simulink model "multimodecbf"  (R2025b)
settings: Solver=FixedStepAuto  StartTime=0.0  StopTime=inf  FixedStep=0.05  RelTol=1e-3
libraries: robotlib x14
settings Model: Creator=sprinkle  LastModifiedBy=sanborkl
settings OptimizationCC: DefaultParameterBehavior=Inlined  EnhancedBackFolding=on  PassReuseOutputArgsAs=Individual arguments  ZeroExternalMemoryAtStartup=off  ZeroInternalMemoryAtStartup=off  MaxStackSize=64  OptimizeBlockOrder=speed  DifferentSizesBufferReuse=on  OptimizationCustomize=off  EfficientTunableParamExpr=on
settings DebuggingCC: ParameterTunabilityLossMsg=error
settings HardwareCC: ProdBitPerPointer=32.0  ProdBitPerSizeT=32.0  ProdBitPerPtrDiffT=32.0  ProdLargestAtomicFloat=None  ProdIntDivRoundTo=Undefined  ProdEndianess=Unspecified  ProdWordSize=32.0  ProdHWDeviceType=Generic->Unspecified (assume 32-bit Generic)
settings SFSimCC: MATLABDynamicMemAlloc=off
settings RTWCC: SystemTargetFile=ert.tlc  HardwareBoard=Robot Operating System (ROS)  TLCOptions="-aInlineSetEventsForThisBaseRateFcn=TLC_FALSE -aSuppressMultiTaskScheduler=TLC_FALSE  -aRateBasedStepFcn=0"  GenCodeOnly=on  TemplateMakefile=ert_default_tmf  Toolchain=Catkin  TargetLang=C++  Description=Embedded Coder
settings CodeAppCC: ForceParamTrailComments=on  IgnoreCustomStorageClasses=off  OperatorAnnotations=on  SimulinkDataObjDesc=on  SFDataObjDesc=on  InsertBlockDesc=on

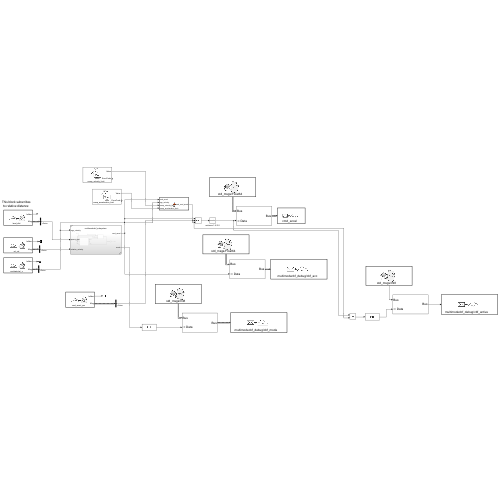
[thumbnail: Simulink's stored preview of the top-level diagram]
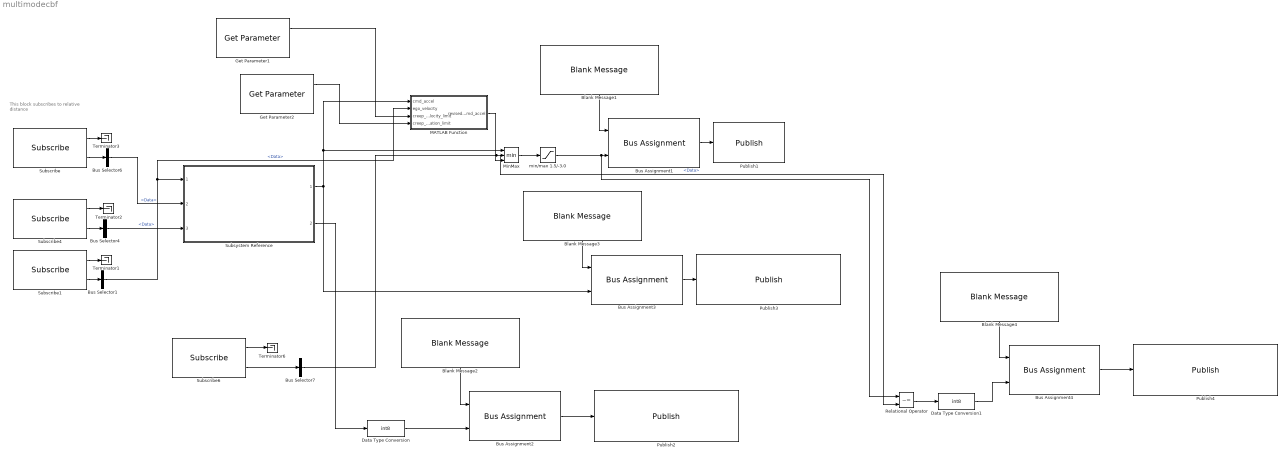
== system multimodecbf ==
  note: This block subscribes
      | to relative distance
  Blank Message1 : robotlib/Blank Message  messageClass=Message  entityType=std_msgs/Float64  messageType=std_msgs/Float64  SampleTime=inf  legacyBusStruct=off
  Blank Message2 : robotlib/Blank Message  messageClass=Message  entityType=std_msgs/Int8  messageType=std_msgs/Int8  SampleTime=inf  legacyBusStruct=off
  Blank Message3 : robotlib/Blank Message  messageClass=Message  entityType=std_msgs/Float64  messageType=std_msgs/Float64  SampleTime=inf  legacyBusStruct=off
  Blank Message4 : robotlib/Blank Message  messageClass=Message  entityType=std_msgs/Int8  messageType=std_msgs/Int8  SampleTime=inf  legacyBusStruct=off
  Bus Assignment{1..4} (4 alike) : BusAssignment  AssignedSignals=Data
  Bus Selector{1,4,6..7} (4 alike) : BusSelector  OutputSignals=Data
  Data Type Conversion : DataTypeConversion  OutDataTypeStr=int8  SaturateOnIntegerOverflow=off  RndMeth=Floor
  Data Type Conversion1 : DataTypeConversion  OutDataTypeStr=int8  SaturateOnIntegerOverflow=off  RndMeth=Floor
  Get Parameter1 : robotlib/Get Parameter  ParameterSource=Specify your own  ParameterName=creep_velocity_limit  ParameterType=double  ParameterMaxArrayLength=16  ParameterInitialValue=0.1  SampleTime=-1  ShowErrorCodeOutput=on  ModelName=multimodecbf  BlockId=ParamGet_multimodecbf_97
  Get Parameter2 : robotlib/Get Parameter  ParameterSource=Specify your own  ParameterName=creep_acceleration_limit  ParameterType=double  ParameterMaxArrayLength=16  ParameterInitialValue=0.0  SampleTime=-1  ShowErrorCodeOutput=on  ModelName=multimodecbf  BlockId=ParamGet_multimodecbf_98
  MATLAB Function : MATLAB Function  TreatAsAtomicUnit=on
  MinMax : MinMax  Inputs=3
  Publish1 : robotlib/Publish  topicSource=Specify your own  topic=cmd_accel  messageType=std_msgs/Float64  legacyBusStruct=off  messageQueueLength=1
  Publish2 : robotlib/Publish  topicSource=Specify your own  topic=multimodecbf_debug/cbf_mode  messageType=std_msgs/Int8  legacyBusStruct=off  messageQueueLength=1
  Publish3 : robotlib/Publish  topicSource=Specify your own  topic=multimodecbf_debug/cbf_acc  messageType=std_msgs/Float64  legacyBusStruct=off  messageQueueLength=1
  Publish4 : robotlib/Publish  topicSource=Specify your own  topic=multimodecbf_debug/cbf_active  messageType=std_msgs/Int8  legacyBusStruct=off  messageQueueLength=1
  Relational Operator : RelationalOperator  Operator=~=  OutDataTypeStr=boolean  RndMeth=Simplest  InputSameDT=off
  Subscribe : robotlib/Subscribe  topicSource=Specify your own  topic=lead_dist  messageType=std_msgs/Float64  SampleTime=-1  legacyBusStruct=off  messageQueueLength=1
  Subscribe1 : robotlib/Subscribe  topicSource=Specify your own  topic=car/state/vel_x  messageType=std_msgs/Float64  SampleTime=-1  legacyBusStruct=off  messageQueueLength=1
  Subscribe4 : robotlib/Subscribe  topicSource=Specify your own  topic=rel_vel  messageType=std_msgs/Float64  SampleTime=-1  legacyBusStruct=off  messageQueueLength=1
  Subscribe6 : robotlib/Subscribe  topicSource=Specify your own  topic=cmd_accel_pre  messageType=std_msgs/Float64  SampleTime=-1  legacyBusStruct=off  messageQueueLength=1
  Subsystem Reference : Subsystem  ReferencedSubsystem=multimodecbf_subsystem
  Terminator{1..3,6} (4 alike) : Terminator
  min/max 1.5/-3.0 : Saturate  UpperLimit=1.5  LowerLimit=-3.0
  wires:
  Bus Assignment1/1 -> Publish1/1
  Bus Selector4/1 -> Subsystem Reference/3  "<Data>"
  Subscribe1/2 -> Bus Selector1/1
  Bus Selector1/1 -> MATLAB Function/2(ego_velocity), Subsystem Reference/1  "<Data>"
  Subscribe4/2 -> Bus Selector4/1
  Bus Selector6/1 -> Subsystem Reference/2  "<Data>"
  Subscribe/2 -> Bus Selector6/1
  Bus Selector7/1 -> Relational Operator/2, MinMax/2  "<Data>"
  Subscribe1/1 -> Terminator1/1
  min/max 1.5/-3.0/1 -> Relational Operator/1, Bus Assignment1/2
  Subscribe6/1 -> Terminator6/1
  Subscribe4/1 -> Terminator2/1
  Subscribe/1 -> Terminator3/1
  Subscribe6/2 -> Bus Selector7/1
  Blank Message1/1 -> Bus Assignment1/1
  Bus Assignment2/1 -> Publish2/1
  Blank Message2/1 -> Bus Assignment2/1
  Blank Message3/1 -> Bus Assignment3/1
  Bus Assignment3/1 -> Publish3/1
  Get Parameter1/1 -> MATLAB Function/3(creep_velocity_limit)
  Get Parameter2/1 -> MATLAB Function/4(creep_acceleration_limit)
  Subsystem Reference/1 -> MinMax/1, MATLAB Function/1(cmd_accel), Bus Assignment3/2
  Subsystem Reference/2 -> Data Type Conversion/1
  Data Type Conversion/1 -> Bus Assignment2/2
  MinMax/1 -> min/max 1.5/-3.0/1
  MATLAB Function/1(revised_cmd_accel) -> MinMax/3
  Relational Operator/1 -> Data Type Conversion1/1
  Blank Message4/1 -> Bus Assignment4/1
  Data Type Conversion1/1 -> Bus Assignment4/2
  Bus Assignment4/1 -> Publish4/1

== matlab function multimodecbf/MATLAB Function ==
  data: cmd_accel input; revised_cmd_accel output; ego_velocity input; creep_velocity_limit input; creep_acceleration_limit input
function revised_cmd_accel = fcn(cmd_accel, ego_velocity, creep_velocity_limit, creep_acceleration_limit)

if (ego_velocity <= creep_velocity_limit) && (cmd_accel <= creep_acceleration_limit)
    revised_cmd_accel = -1;
else
    revised_cmd_accel = cmd_accel;
end
